simulink model "ml_project"  (R2025b)
settings: Solver=VariableStepAuto  StartTime=0.0  StopTime=10000  RelTol=1e-3
undefined symbols (not defined in the file): Day_in_val, Hour_in_val, Season_in_val
settings Model: Creator=lenovo  LastModifiedBy=lenovo

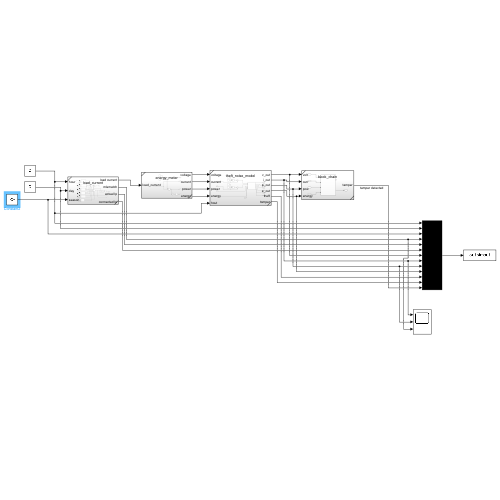
[thumbnail: Simulink's stored preview of the top-level diagram]
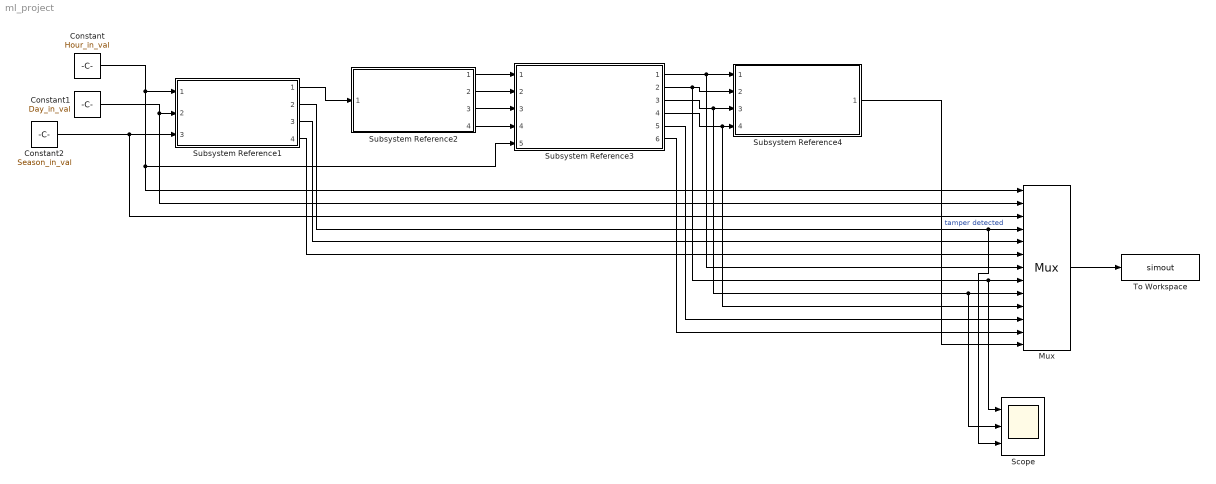
== system ml_project ==
  Constant : Constant  Value=Hour_in_val
  Constant1 : Constant  Value=Day_in_val
  Constant2 : Constant  Value=Season_in_val
  Mux : Mux  Inputs=13
  Scope : Scope  NumInputPorts=3
  Subsystem Reference1 : Subsystem  ReferencedSubsystem=load_current
  Subsystem Reference2 : Subsystem  ReferencedSubsystem=energy_meter
  Subsystem Reference3 : Subsystem  ReferencedSubsystem=theft_noise_model
  Subsystem Reference4 : Subsystem  ReferencedSubsystem=block_chain
  To Workspace : ToWorkspace  VariableName=simout  SampleTime=-1
  wires:
  Constant/1 -> Subsystem Reference1/1, Mux/1, Subsystem Reference3/5
  Constant1/1 -> Mux/2, Subsystem Reference1/2
  Constant2/1 -> Mux/3, Subsystem Reference1/3
  Subsystem Reference1/1 -> Subsystem Reference2/1
  Subsystem Reference2/1 -> Subsystem Reference3/1
  Subsystem Reference2/2 -> Subsystem Reference3/2
  Subsystem Reference2/3 -> Subsystem Reference3/3
  Subsystem Reference2/4 -> Subsystem Reference3/4
  Subsystem Reference3/1 -> Mux/7, Subsystem Reference4/1
  Subsystem Reference3/4 -> Mux/10, Subsystem Reference4/4
  Subsystem Reference3/3 -> Scope/2, Mux/9, Subsystem Reference4/3
  Subsystem Reference3/2 -> Scope/1, Mux/8, Subsystem Reference4/2
  Subsystem Reference1/2 -> Scope/3, Mux/4
  Subsystem Reference1/3 -> Mux/5
  Subsystem Reference1/4 -> Mux/6
  Subsystem Reference3/5 -> Mux/11
  Subsystem Reference3/6 -> Mux/12
  Subsystem Reference4/1 -> Mux/13  "tamper detected"
  Mux/1 -> To Workspace/1
